simulink model "nonlinearCossanddeadtimeDAB"  (R2024b)
settings: Solver=ode23t  StartTime=0.0  StopTime=0.1  FixedStep=Tsolver  MaxStep=Tsolver  RelTol=1e-05
values from neighbouring files (symbols this model uses):
  f_sw = 20e3    (= 20000)    [zvs_init.m]
  PD_S1 = PD(1)    [zvs_init.m]
  PD_S2 = PD(2)    [zvs_init.m]
  PD_S3 = PD(3)    [zvs_init.m]
  PD_S4 = PD(4)    [zvs_init.m]
  PD_S5 = PD(5)    [zvs_init.m]
  PD_S6 = PD(6)    [zvs_init.m]
  PD_S7 = PD(7)    [zvs_init.m]
  PD_S8 = PD(8)    [zvs_init.m]
  PW_PCT = 100*(0.5 - tdead*f_sw)    (= 49.6)    [zvs_init.m]
  Ri = 0.1    [zvs_init.m]
  Ro = 0.1    [zvs_init.m]
  Rs = 25e-3    (= 0.025)    [zvs_init.m]
  Vi = 800    [zvs_init.m]
  Vo = 800    [zvs_init.m]
libraries: fl_lib x21, nesl_utility x19, zvslib_lib x8, ee_lib x8
settings Model: Creator=amina  LastModifiedBy=amina
settings SolverCC: MaxConsecutiveMinStep=100
settings DataIOCC: SaveOutput=off  SignalLogging=off  DSMLogging=off  SaveTime=off  ReturnWorkspaceOutputsName=out_analytic

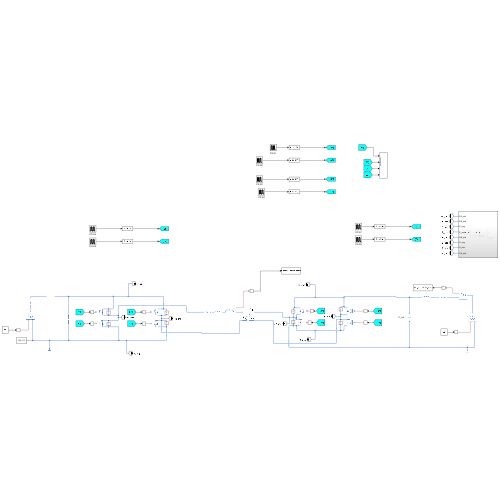
[thumbnail: Simulink's stored preview of the top-level diagram]
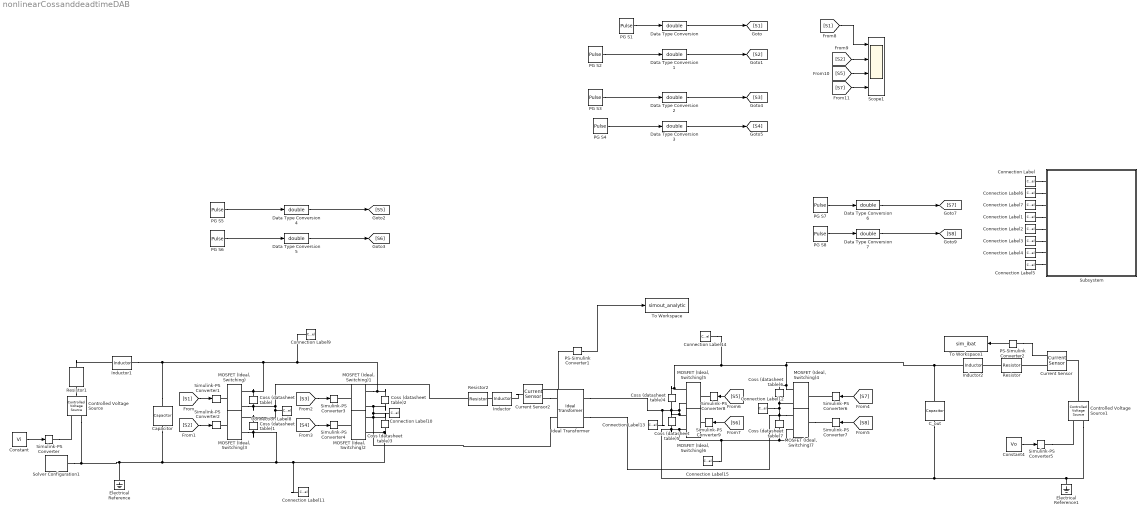
== system nonlinearCossanddeadtimeDAB ==
  C_out : fl_lib/Electrical/Electrical Elements/Capacitor  c=Co F  r=0 Ohm  g=0 1/Ohm  i_specify=off  i_priority=None  i=0 A  i_nominal_specify=off  i_nominal_value=1  i_nominal_unit=A  v_specify=off  v_priority=None  v=0 V  v_nominal_specify=off  v_nominal_value=1  v_nominal_unit=V  vc_specify=off  vc_priority=High  vc=V_cap_init V  vc_nominal_specify=off  vc_nominal_value=1  vc_nominal_unit=V
  Capacitor : fl_lib/Electrical/Electrical Elements/Capacitor  c=Ci F  r=1e-6 Ohm  g=0 1/Ohm  i_specify=off  i_priority=None  i=0 A  i_nominal_specify=off  i_nominal_value=1  i_nominal_unit=A  v_specify=off  v_priority=None  v=0 V  v_nominal_specify=off  v_nominal_value=1  v_nominal_unit=V  vc_specify=off  vc_priority=High  vc=V_cap_init V  vc_nominal_specify=off  vc_nominal_value=1  vc_nominal_unit=V
  Connection Label : ConnectionLabel  Label=PA_mid
  Connection Label1 : ConnectionLabel  Label=P_pos
  Connection Label10 : ConnectionLabel  Label=PB_mid
  Connection Label11 : ConnectionLabel  Label=P_neg
  Connection Label12 : ConnectionLabel  Label=SB_mid
  Connection Label13 : ConnectionLabel  Label=SA_mid
  Connection Label14 : ConnectionLabel  Label=S_pos
  Connection Label15 : ConnectionLabel  Label=S_neg
  Connection Label2 : ConnectionLabel  Label=SB_mid
  Connection Label3 : ConnectionLabel  Label=S_neg
  Connection Label4 : ConnectionLabel  Label=S_pos
  Connection Label5 : ConnectionLabel  Label=SA_mid
  Connection Label6 : ConnectionLabel  Label=PB_mid
  Connection Label7 : ConnectionLabel  Label=P_neg
  Connection Label8 : ConnectionLabel  Label=PA_mid
  Connection Label9 : ConnectionLabel  Label=P_pos
  Constant : Constant  Value=Vi
  Constant4 : Constant  Value=Vo
  Controlled Voltage Source : fl_lib/Electrical/Electrical Sources/Controlled Voltage Source
  Controlled Voltage Source1 : fl_lib/Electrical/Electrical Sources/Controlled Voltage Source
  Coss (datasheet table){,1..7} (8 alike) : zvslib_lib/Coss (datasheet table)  Vtab=COSS_V V  Ctab=COSS_C F  i_specify=off  i_priority=None  i=0 A  i_nominal_specify=off  i_nominal_value=1  i_nominal_unit=A  v_specify=off  v_priority=None  v=0 V  v_nominal_specify=off  v_nominal_value=1  v_nominal_unit=V
      settings: InternalSimscapePortConfiguration="{\"Bottom\":[],\"Left\":[{\"id\":\"p\",\"label\":\"+\",\"type\":\"foundation.electrical.electrical\"}],\"Right\":[{\"id\":\"n\",\"label\":\"-\",\"type\":\"foundation.electrical.electrical\"}],\"Top\":[]}"
  Current Sensor : fl_lib/Electrical/Electrical Sensors/Current Sensor
  Current Sensor2 : fl_lib/Electrical/Electrical Sensors/Current Sensor
  Data Type Conversion{,1..7} (8 alike) : DataTypeConversion  OutDataTypeStr=double  SaturateOnIntegerOverflow=off  RndMeth=Floor
  Electrical Reference : fl_lib/Electrical/Electrical Elements/Electrical Reference
  Electrical Reference1 : fl_lib/Electrical/Electrical Elements/Electrical Reference
  Ideal Transformer : fl_lib/Electrical/Electrical Elements/Ideal Transformer  n=n  i1_specify=off  i1_priority=None  i1=0 A  i1_nominal_specify=off  i1_nominal_value=1  i1_nominal_unit=A  v1_specify=off  v1_priority=None  v1=0 V  v1_nominal_specify=off  v1_nominal_value=1  v1_nominal_unit=V  i2_specify=off  i2_priority=None  i2=0 A  i2_nominal_specify=off  i2_nominal_value=1  i2_nominal_unit=A  v2_specify=off  v2_priority=None  v2=0 V  v2_nominal_specify=off  v2_nominal_value=1  v2_nominal_unit=V
  Inductor : fl_lib/Electrical/Electrical Elements/Inductor  l=Ls H  r=0 Ohm  g=1e-9 1/Ohm  i_specify=off  i_priority=None  i=0 A  i_nominal_specify=off  i_nominal_value=1  i_nominal_unit=A  v_specify=off  v_priority=None  v=0 V  v_nominal_specify=off  v_nominal_value=1  v_nominal_unit=V  i_L_specify=off  i_L_priority=High  i_L=0 A  i_L_nominal_specify=off  i_L_nominal_value=1  i_L_nominal_unit=A
  Inductor1 : fl_lib/Electrical/Electrical Elements/Inductor  l=Li H  r=0 Ohm  g=1e-9 1/Ohm  i_specify=off  i_priority=None  i=0 A  i_nominal_specify=off  i_nominal_value=1  i_nominal_unit=A  v_specify=off  v_priority=None  v=0 V  v_nominal_specify=off  v_nominal_value=1  v_nominal_unit=V  i_L_specify=off  i_L_priority=High  i_L=0 A  i_L_nominal_specify=off  i_L_nominal_value=1  i_L_nominal_unit=A
  Inductor2 : fl_lib/Electrical/Electrical Elements/Inductor  l=Lo H  r=0 Ohm  g=1e-9 1/Ohm  i_specify=off  i_priority=None  i=0 A  i_nominal_specify=off  i_nominal_value=1  i_nominal_unit=A  v_specify=off  v_priority=None  v=0 V  v_nominal_specify=off  v_nominal_value=1  v_nominal_unit=V  i_L_specify=off  i_L_priority=High  i_L=0 A  i_L_nominal_specify=off  i_L_nominal_value=1  i_L_nominal_unit=A
  MOSFET (Ideal, Switching){,1..7} (8 alike) : ee_lib/Semiconductors & Converters/MOSFET (Ideal, Switching)  port_option=ee.enum.controlport.ps  Rds=Rds Ohm  Goff=G_mosfet 1/Ohm  Vth=Vth V  diode_param=ee.enum.semiconductors.protectionDiode.nodynamics  diode_Vf=Vf_diode V  diode_Ron=0.001 Ohm  diode_Goff=1e-5 1/Ohm  diode_C=50e-9 F  diode_iRM=-235 A  diode_iF=300 A  diode_idot=-50 A/us  diode_trr_param=ee.enum.converters.diodeReverseParam.trr_factor  diode_trr_factor=3  diode_trr=15 us  diode_Qrr=1500 s*uA  ids_specify=off  ids_priority=None  ids=0 A  ids_nominal_specify=off  ids_nominal_value=1  ids_nominal_unit=A  vds_specify=off  vds_priority=None  vds=0 V  vds_nominal_specify=off  vds_nominal_value=1  vds_nominal_unit=V  vgs_specify=off  vgs_priority=None  vgs=0 V  vgs_nominal_specify=off  vgs_nominal_value=1  vgs_nominal_unit=V  thermal_loss_option=ee.enum.converters.thermalLossOption.constantvalues  Von_data=[0, 1.8, 3.2, 6, 10, 16; 0, 2, 5.5, 9.5, 15, 25] V  Tj=[298.15, 448.15] K  Iout_data=[0, 20, 40, 60, 80, 100] A  Eon_data=[0, 55.04, 124.57, 235.53, 362.12; 0, 71.25, 161.25, 304.88, 468.75] * 1e-6 J  Eoff_data=[0, 18, 30, 56.1, 76.5; 0, 22.5, 37.5, 70.13, 95.63] * 1e-6 J  Eon_data_3D=[zeros(2, 5, 3)] J  Eoff_data_3D=[zeros(2, 5, 3)] J  Tj_loss=[298.15, 448.15] K  Iout_data_loss=[0, 10, 20, 30, 40] A  tabulateWithVds=false  Vds_loss=[0, 150, 300] V  Eon_scalar=22.86e-3 J  Eoff_scalar=17.14e-3 J  Voff=300 V  Iout_scalar=600 A  useCurrentFromPreviousCycle=false  useVoltageFromPreviousCycle=false  diodeModelType=ee.enum.converters.diodeModelType.pwl  diodeTableType=ee.enum.diode.tableType.IfMat  diode_ReverseIVType=ee.enum.diode.diodeReverseIV.constant  diode_IfMat=[.07, .12, .19, 1.75, 4.24, 7.32, 11.2; .16, .3, .72, 2.14, 4.02, 6.35, 9.12] A  diode_VfMat=[.9, 1.15, 1.25, 1.5, 1.75, 2.17, 2.6, 2.85; .58, .68, .75, 1.1, 1.38, 1.77, 2.27, 2.7] V  diode_TjVec=[25, 125] degC  diode_VfVec=[.5, .7, .9, 1.3, 1.7, 2.1, 2.5] V  diode_IfVec=[.1, .2, .5, 1, 2, 4, 7, 10] A  diode_IrMat=[1e-06, 2e-06, 5e-06, 1e-05, 2.5e-05, 5e-05, .0001; 2e-06, 5e-06, 1e-05, 4e-05, 8e-05, .0002, .0005] A  diode_VrMat=[10, 100, 200, 250, 300, 325, 350; 10, 70, 160, 220, 270, 300, 320] V  diode_VrVec=[10, 20, 40, 50, 70, 80, 100] V  diode_IrVec=[1e-06, 2e-06, 5e-06, 1e-05, 2e-05, 5e-05, .0001] A  diode_Vr=-600 V  diode_Ls=150 nH  diode_Erec=0.03 J  diode_rec_loss_model=ee.enum.diode.reverseRecoveryModel.fixed  diode_ErecVal=0 J  diode_scaleWithIandV=true  diode_ErecMat=zeros(2, 3) J  diode_TjrecVec=[298.15, 398.15] K  diode_IfrecVec=[.1, 1, 10] A  diode_IrecVal=10 A  diode_VrecVal=10 V  diode_tFilter=1 / 1000 / 100 s  separateThermalPortForDiode=false  thermal_network_parameterization=ee.enum.thermalNetworkTopology.external  Rth=[.03, .2] K/W  Rth_Cauer=[.03, .1, .2] K/W  Rth_Foster=[.08, .14, .22, .16] K/W  thermal_mass_parameterization=ee.enum.thermalNetwork.timeconstant  thermal_mass=[3, 25] J/K  thermal_mass_Cauer=[3, 10, 25] J/K  thermal_mass_Foster=[.001, .005, .05, .5] J/K  thermal_time_constant=[.1, 5] s  thermal_time_constant_Cauer=[.1, 1, 5] s  thermal_time_constant_Foster=[7e-05, .0007, .01, .08] s  thermal_mass_initial_temperatures=[25, 25] degC  thermal_mass_initial_temperatures_Cauer=[25, 25, 25] degC  junction_thermal_mass=0.1 J/K  Tvec_initial_Foster=[25, 25, 25, 25] degC  RthDiode=[.03, .2] K/W  RthCauerDiode=[.03, .1, .2] K/W  RthFosterDiode=[.03, .2] K/W  thermalMassDiode=[3, 25] J/K  thermalMassCauerDiode=[3, 10, 25] J/K  thermalMassFosterDiode=[33, 50] J/K  thermalTauDiode=[.1, 5] s  thermalTauCauerDiode=[.1, 1, 5] s  thermalTauFosterDiode=[1, 10] s  thermalMassInitTempDiode=[25, 25] degC  thermalMassInitTempCauerDiode=[25, 25, 25] degC  junctionthermalMassDiode=0.1 J/K  TVecInitialFosterDiode=[25, 25, 25, 25] degC  no_thermal_network=0  mosfet_junction_temperature_specify=off  mosfet_junction_temperature_priority=None  mosfet_junction_temperature=25 degC  mosfet_junction_temperature_nominal_specify=off  mosfet_junction_temperature_nominal_value=1  mosfet_junction_temperature_nominal_unit=degC  diode_junction_temperature_specify=off  diode_junction_temperature_priority=None  diode_junction_temperature=25 degC  diode_junction_temperature_nominal_specify=off  diode_junction_temperature_nominal_value=1  diode_junction_temperature_nominal_unit=degC  Qj_specify=off  Qj_priority=None  Qj=0 W  Qj_nominal_specify=off  Qj_nominal_value=1  Qj_nominal_unit=W  accumulatedSwitchingLosses_specify=off  accumulatedSwitchingLosses_priority=None  accumulatedSwitchingLosses=0 J
  PG S1 : DiscretePulseGenerator  PulseType=Time based  Period=1/f_sw  PulseWidth=PW_PCT  PhaseDelay=PD_S1
  PG S2 : DiscretePulseGenerator  PulseType=Time based  Period=1/f_sw  PulseWidth=PW_PCT  PhaseDelay=PD_S2
  PG S3 : DiscretePulseGenerator  PulseType=Time based  Period=1/f_sw  PulseWidth=PW_PCT  PhaseDelay=PD_S3
  PG S4 : DiscretePulseGenerator  PulseType=Time based  Period=1/f_sw  PulseWidth=PW_PCT  PhaseDelay=PD_S4
  PG S5 : DiscretePulseGenerator  PulseType=Time based  Period=1/f_sw  PulseWidth=PW_PCT  PhaseDelay=PD_S5
  PG S6 : DiscretePulseGenerator  PulseType=Time based  Period=1/f_sw  PulseWidth=PW_PCT  PhaseDelay=PD_S6
  PG S7 : DiscretePulseGenerator  PulseType=Time based  Period=1/f_sw  PulseWidth=PW_PCT  PhaseDelay=PD_S7
  PG S8 : DiscretePulseGenerator  PulseType=Time based  Period=1/f_sw  PulseWidth=PW_PCT  PhaseDelay=PD_S8
  PS-Simulink Converter1 : nesl_utility/PS-Simulink Converter  PhysicalDomain=network_engine_domain  SubClassName=ps_output  LeftPortType=input  RightPortType=output  PseudoPeriodic=off  Frequencies=[]  VectorFormat=inherit  Unit=inherit  AffineConversion=off
  PS-Simulink Converter2 : nesl_utility/PS-Simulink Converter  PhysicalDomain=network_engine_domain  SubClassName=ps_output  LeftPortType=input  RightPortType=output  PseudoPeriodic=off  Frequencies=[]  VectorFormat=inherit  Unit=A  AffineConversion=off
  Resistor : fl_lib/Electrical/Electrical Elements/Resistor  R=Ro Ohm  i_specify=off  i_priority=None  i=0 A  i_nominal_specify=off  i_nominal_value=1  i_nominal_unit=A  v_specify=off  v_priority=None  v=0 V  v_nominal_specify=off  v_nominal_value=1  v_nominal_unit=V
  Resistor1 : fl_lib/Electrical/Electrical Elements/Resistor  R=Ri Ohm  i_specify=off  i_priority=None  i=0 A  i_nominal_specify=off  i_nominal_value=1  i_nominal_unit=A  v_specify=off  v_priority=None  v=0 V  v_nominal_specify=off  v_nominal_value=1  v_nominal_unit=V
  Resistor2 : fl_lib/Electrical/Electrical Elements/Resistor  R=Rs Ohm  i_specify=off  i_priority=None  i=0 A  i_nominal_specify=off  i_nominal_value=1  i_nominal_unit=A  v_specify=off  v_priority=None  v=0 V  v_nominal_specify=off  v_nominal_value=1  v_nominal_unit=V
  Scope1 : Scope  NumInputPorts=4
  Simulink-PS Converter{,1..9} (10 alike) : nesl_utility/Simulink-PS Converter  PhysicalDomain=network_engine_domain  SubClassName=ps_input  LeftPortType=input  RightPortType=output  PseudoPeriodic=off  Frequencies=[]  NoiseDistribution=none  NoiseParameters=[]  Unit=1  AffineConversion=off  FilteringAndDerivatives=provide  SimscapeFilterOrder=1  InputFilterTimeConstant=0.001  UdotUserProvided=0
  Solver Configuration1 : nesl_utility/Solver Configuration  PhysicalDomain=network_engine_domain  SubClassName=solver  LeftPortType=input  RightPortType=generic  Tones=[]  Harmonics=[]  SimulateNoise=off  Profile=off  UseLocalSampling=off  EnableSwitchedLinearOptims=on  FrequencyDomain=off  UseCCode=off  RelTol=0.001  AbsTol=1e-06  MinStep=1e-09  ToWorkspace=off  RevertToSquareIcSolve=off  NumHomotopyIterations=100  PhasorMode=off  PhasorModeNumHarmonics=1  ConsistencySolver=NEWTON_FTOL  IndexReductionMethod=DerivativeReplacement  DoDC=off  ResidualTolerance=1e-09  ConsistencyTolSource=GLOBAL  ConsistencyAbsTol=0.001  ConsistencyRelTol=0.001  ConsistencyTolFactor=0.001  UseLocalSolver=off  LocalSolverChoice=NE_BACKWARD_EULER_ADVANCER  ResolveIndetEquations=on  FunctionEvalNumThread=1  LocalSolverSampleTime=0.001  DoFixedCost=off  MaxNonlinIter=3  MaxModeIter=2  ComputeImpulses=off  ImpulseIterations=2  LinearAlgebra=auto  LinearAlgebraNumThread=0  EquationFormulation=NE_TIME_EF  DelaysMemoryBudget=1024  AutomaticFiltering=on  FilteringTimeConstant=0.001  PartitionStorageMethod=AS_NEEDED  PartitionMemoryBudget=1024  PartitionMethod=ROBUST  MultibodyUseLocalSolver=off  MultibodyLocalSolverChoice=ODE1  MultibodyLocalSolverSampleTime=0.001
  Subsystem : Subsystem
  To Workspace : ToWorkspace  VariableName=simout_analytic  SaveFormat=Timeseries  SampleTime=-1
  To Workspace1 : ToWorkspace  VariableName=sim_ibat  SaveFormat=Timeseries  SampleTime=-1
  wires:
  Data Type Conversion/1 -> [S1]
  Constant/1 -> Simulink-PS Converter/1
  [S1] -> Scope1/1
  [S2] -> Scope1/2
  [S3] -> Simulink-PS Converter3/1
  [S4] -> Simulink-PS Converter4/1
  [S1] -> Simulink-PS Converter1/1
  [S6] -> Simulink-PS Converter9/1
  [S7] -> Scope1/4
  [S7] -> Simulink-PS Converter6/1
  Data Type Conversion6/1 -> [S7]
  Data Type Conversion4/1 -> [S5]
  Data Type Conversion1/1 -> [S2]
  Data Type Conversion7/1 -> [S8]
  Data Type Conversion5/1 -> [S6]
  [S5] -> Scope1/3
  Data Type Conversion3/1 -> [S4]
  [S2] -> Simulink-PS Converter2/1
  Data Type Conversion2/1 -> [S3]
  PS-Simulink Converter1/1 -> To Workspace/1
  [S5] -> Simulink-PS Converter8/1
  [S8] -> Simulink-PS Converter7/1
  Constant4/1 -> Simulink-PS Converter5/1
  PS-Simulink Converter2/1 -> To Workspace1/1
  PG S1/1 -> Data Type Conversion/1
  PG S2/1 -> Data Type Conversion1/1
  PG S3/1 -> Data Type Conversion2/1
  PG S4/1 -> Data Type Conversion3/1
  PG S5/1 -> Data Type Conversion4/1
  PG S8/1 -> Data Type Conversion7/1
  PG S7/1 -> Data Type Conversion6/1
  PG S6/1 -> Data Type Conversion5/1
  connections:
  Controlled Voltage Source/RConn2 -- Solver Configuration1/RConn1 -- Electrical Reference/LConn1 -- Coss (datasheet table)1/RConn1 -- "MOSFET (Ideal, Switching)3"/RConn2 -- Connection Label11/LConn1 -- "MOSFET (Ideal, Switching)2"/RConn2 -- Coss (datasheet table)3/RConn1 -- Capacitor/RConn1
  Capacitor/LConn1 -- Connection Label9/LConn1 -- "MOSFET (Ideal, Switching)1"/RConn1 -- Coss (datasheet table)2/LConn1 -- Coss (datasheet table)/LConn1 -- "MOSFET (Ideal, Switching)"/RConn1 -- Inductor1/RConn1
  C_out/RConn1 -- Controlled Voltage Source1/RConn2 -- Electrical Reference1/LConn1 -- Coss (datasheet table)5/RConn1 -- "MOSFET (Ideal, Switching)7"/RConn2 -- Coss (datasheet table)7/RConn1 -- Connection Label15/LConn1 -- "MOSFET (Ideal, Switching)6"/RConn2
  Resistor2/RConn1 -- Connection Label8/LConn1 -- Coss (datasheet table)1/LConn1 -- "MOSFET (Ideal, Switching)3"/RConn1 -- Coss (datasheet table)/RConn1 -- "MOSFET (Ideal, Switching)"/RConn2
  "MOSFET (Ideal, Switching)1"/RConn2 -- Coss (datasheet table)2/RConn1 -- Connection Label10/LConn1 -- "MOSFET (Ideal, Switching)2"/RConn1 -- Ideal Transformer/LConn2 -- Coss (datasheet table)3/LConn1
  Inductor2/LConn1 -- C_out/LConn1 -- Connection Label14/LConn1 -- Coss (datasheet table)4/LConn1 -- "MOSFET (Ideal, Switching)5"/RConn1 -- Coss (datasheet table)6/LConn1 -- "MOSFET (Ideal, Switching)4"/RConn1
  "MOSFET (Ideal, Switching)5"/RConn2 -- Connection Label13/LConn1 -- Ideal Transformer/RConn1 -- Coss (datasheet table)4/RConn1 -- Coss (datasheet table)5/LConn1 -- "MOSFET (Ideal, Switching)6"/RConn1
  "MOSFET (Ideal, Switching)7"/RConn1 -- Coss (datasheet table)7/LConn1 -- Ideal Transformer/RConn2 -- Coss (datasheet table)6/RConn1 -- "MOSFET (Ideal, Switching)4"/RConn2 -- Connection Label12/LConn1
  Simulink-PS Converter5/RConn1 -- Controlled Voltage Source1/RConn1
  Simulink-PS Converter6/RConn1 -- "MOSFET (Ideal, Switching)4"/LConn1
  Current Sensor2/LConn1 -- Inductor/RConn1
  Simulink-PS Converter/RConn1 -- Controlled Voltage Source/RConn1
  Resistor2/LConn1 -- Inductor/LConn1
  Resistor1/RConn1 -- Controlled Voltage Source/LConn1
  PS-Simulink Converter1/LConn1 -- Current Sensor2/RConn1
  "MOSFET (Ideal, Switching)1"/LConn1 -- Simulink-PS Converter3/RConn1
  Current Sensor2/RConn2 -- Ideal Transformer/LConn1
  "MOSFET (Ideal, Switching)3"/LConn1 -- Simulink-PS Converter2/RConn1
  "MOSFET (Ideal, Switching)2"/LConn1 -- Simulink-PS Converter4/RConn1
  "MOSFET (Ideal, Switching)7"/LConn1 -- Simulink-PS Converter7/RConn1
  Simulink-PS Converter1/RConn1 -- "MOSFET (Ideal, Switching)"/LConn1
  Resistor1/LConn1 -- Inductor1/LConn1
  Resistor/RConn1 -- Inductor2/RConn1
  Simulink-PS Converter8/RConn1 -- "MOSFET (Ideal, Switching)5"/LConn1
  Simulink-PS Converter9/RConn1 -- "MOSFET (Ideal, Switching)6"/LConn1
  Connection Label3/LConn1 -- Subsystem/LConn6
  Connection Label/LConn1 -- Subsystem/LConn1
  Connection Label7/LConn1 -- Subsystem/LConn3
  Connection Label2/LConn1 -- Subsystem/LConn5
  Connection Label5/LConn1 -- Subsystem/LConn8
  Connection Label6/LConn1 -- Subsystem/LConn2
  Connection Label1/LConn1 -- Subsystem/LConn4
  Connection Label4/LConn1 -- Subsystem/LConn7
  Current Sensor/RConn2 -- Resistor/LConn1
  Controlled Voltage Source1/LConn1 -- Current Sensor/LConn1
  PS-Simulink Converter2/LConn1 -- Current Sensor/RConn1

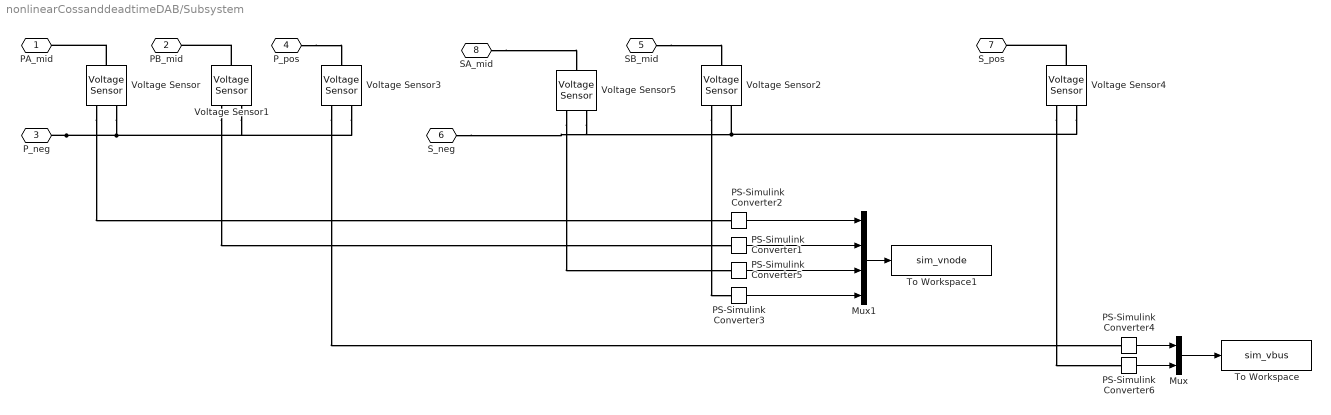
== system nonlinearCossanddeadtimeDAB/Subsystem ==
  Mux : Mux  Inputs=2
  Mux1 : Mux
  PS-Simulink Converter{1..6} (6 alike) : nesl_utility/PS-Simulink Converter  PhysicalDomain=network_engine_domain  SubClassName=ps_output  LeftPortType=input  RightPortType=output  PseudoPeriodic=off  Frequencies=[]  VectorFormat=inherit  Unit=V  AffineConversion=off
  To Workspace : ToWorkspace  VariableName=sim_vbus  SaveFormat=Timeseries  SampleTime=-1
  To Workspace1 : ToWorkspace  VariableName=sim_vnode  SaveFormat=Timeseries  SampleTime=-1
  Voltage Sensor{,1..5} (6 alike) : fl_lib/Electrical/Electrical Sensors/Voltage Sensor
  PA_mid : PMIOPort  Side=Left
  PB_mid : PMIOPort  Port=2  Side=Left
  P_neg : PMIOPort  Port=3  Side=Left
  P_pos : PMIOPort  Port=4  Side=Left
  SB_mid : PMIOPort  Port=5  Side=Left
  S_neg : PMIOPort  Port=6  Side=Left
  S_pos : PMIOPort  Port=7  Side=Left
  SA_mid : PMIOPort  Port=8  Side=Left
  wires:
  PS-Simulink Converter2/1 -> Mux1/1
  PS-Simulink Converter1/1 -> Mux1/2
  PS-Simulink Converter5/1 -> Mux1/3
  PS-Simulink Converter3/1 -> Mux1/4
  Mux1/1 -> To Workspace1/1
  PS-Simulink Converter4/1 -> Mux/1
  PS-Simulink Converter6/1 -> Mux/2
  Mux/1 -> To Workspace/1
  connections:
  Voltage Sensor/LConn1 -- PA_mid/RConn1
  P_neg/RConn1 -- Voltage Sensor/RConn2 -- Voltage Sensor3/RConn2 -- Voltage Sensor1/RConn2
  Voltage Sensor1/LConn1 -- PB_mid/RConn1
  Voltage Sensor4/RConn2 -- Voltage Sensor2/RConn2 -- S_neg/RConn1 -- Voltage Sensor5/RConn2
  SB_mid/RConn1 -- Voltage Sensor2/LConn1
  P_pos/RConn1 -- Voltage Sensor3/LConn1
  Voltage Sensor4/LConn1 -- S_pos/RConn1
  Voltage Sensor/RConn1 -- PS-Simulink Converter2/LConn1
  Voltage Sensor1/RConn1 -- PS-Simulink Converter1/LConn1
  SA_mid/RConn1 -- Voltage Sensor5/LConn1
  Voltage Sensor5/RConn1 -- PS-Simulink Converter5/LConn1
  Voltage Sensor2/RConn1 -- PS-Simulink Converter3/LConn1
  Voltage Sensor3/RConn1 -- PS-Simulink Converter4/LConn1
  Voltage Sensor4/RConn1 -- PS-Simulink Converter6/LConn1
